simulink model "Task 2 – Battery Modeling"  (R2025b)
settings: Solver=ode23tb  StartTime=0.0  StopTime=35  RelTol=5e-3
model workspace (MAT data in the model file):
  Eng.Tbts = [18.9199441202 18.9199441202 24.2934146345 29.2101064979 38.0525747067 43.75 43.7497238015 43.7499913003 43.75 43.75 43.75 43.75 43.75 39.375 35 30.625]
  Eng.Nbts = [0 1500 2107.14285714 2714.28571429 3321.42857143 3928.57142857 4535.71428571 5142.85714286 5750 6357.14285714 6964.28571429 7571.42857143 8178.57142857 8785.71428571 9392.85714286 10000]
  Nmtr = 18.5
  SteerLim = 60
  TrackPoints = [-15 -12 -9 -6 -3 5.58745102111e-16 2.81978007367 5.36354042717 7.38228007367 8.67839071119 9.125 8.67839071119 ... (270 elements, 90x3)]
  Trans.InputShaftInertia = 0.01
  Trans.InputShaftDamping = 0.001
  Trans.FinalDrive = 3.25
  Trans.GearRatios = [-3.82 4.56 4.56 3.385 2.857 2.444 2 1]
  Trans.GearNums = [-1 0 1 2 3 4 5 6]
  Trans.Inertias = [0.032 0.007 0.032 0.025 0.0155 0.007 0.0025 0.0025]
  Trans.DampingCoeffs = [0.003 0.001 0.003 0.0025 0.002 0.001 0.001 0.001]
  Trans.Efficiencies = [0.9 0.9 0.9 0.9 0.9 0.95 0.95 0.95]
  Trans.ShiftTau = 0.02
  Ts = 0.02
  VEH.Mass = 230
  VEH.StaticNormalFrontLoad.FR = 575
  VEH.StaticNormalFrontLoad.FL = 575
  VEH.StaticNormalRearLoad.RR = 575
  VEH.StaticNormalRearLoad.RL = 322
  VEH.WheelBase = 1.7
  VEH.FrontAxlePositionfromCG = 0.75
  VEH.RearAxlePositionfromCG = 0.75
  VEH.HeightCG = 0.25
  VEH.FrontalArea = 2.11
  VEH.DragCoefficient = 0.33
  VEH.NumberOfWheelsPerAxle = 2
  VEH.PitchMomentInertia = 384.533333333
  VEH.RollMomentInertia = 86.4666666667
  VEH.YawMomentInertia = 413.2
  VEH.SteeringRatio = 18
  VEH.TrackWidth = 1.2
  VEH.SprungMass = 210
  VEH.InitialLongPosition = -15
  VEH.InitialLatPosition = 0
  VEH.InitialVertPosition = -0.2
  VEH.InitialRollAngle = 0
  VEH.InitialPitchAngle = 0
  VEH.InitialYawAngle = 0
  VEH.InitialLongVel = 0
  VEH.InitialLatVel = 0
  VEH.InitialVertVel = 0
  VEH.InitialRollRate = 0
  VEH.InitialPitchRate = 0
  VEH.InitialYawRate = 0
undefined symbols (not defined in the file or in its folder): BdyFrm, InertFrm
libraries: autolibsharedcoupling x11, simulink x9, sim3dlib x7, autolibutils x5, autolibshareddiff x5, sim3dautolib x3, vehdynlibtirecommon x3, sharedtransform x3, vehdynlibdriver x2, vehdynlibviscommon x2, vehdynlibtire x1, autolibmappedmotor x1
(part 1 of 4)
settings Model: SimulationMode=accelerator  Creator=The MathWorks, Inc.
settings SolverCC: ZeroCrossAlgorithm=Adaptive
settings OptimizationCC: ReuseModelBlockBuffer=off
settings DebuggingCC: IgnoredZcDiagnostic=none  SubsystemReferenceDiagnosticForUnitTest=warning
settings RTWCC: GPUComputeCapability=3.5

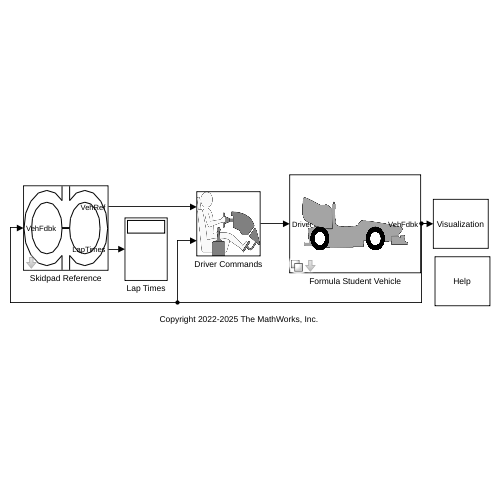
[thumbnail: Simulink's stored preview of the top-level diagram]
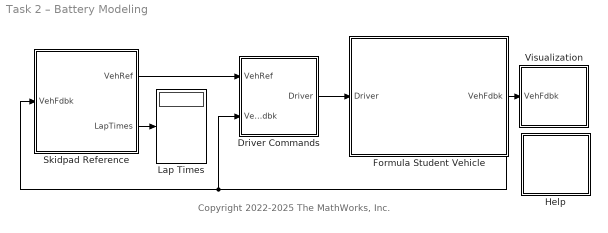
== system Task 2 – Battery Modeling ==
  note: Copyright 2022-2025 The MathWorks, Inc.
  Driver Commands : Subsystem  VariantControl=0
      mask Display: image('driverlatlongshift.png');
  Formula Student Vehicle : Subsystem  Variant=on  VariantControl=Choice  mask(Vehicle Setup){vehType=Simulink Physics}
      mask prompts: vehType "Vehicle Type:"
      mask help:
      | Choose a vehicle with powertrain and vehicle physics from Simulink blocks or one that uses a game engine physics.
      | The model will automatically configure the subsystems and settings to accomodate your choice.
      mask Help: eval('vdynblkshelp(''vdynblksformula'')');
      mask TypeOptions vehType: Game Engine Physics | Simulink Physics
      mask Callback vehType:
      | if strcmp(get_param(gcb,"vehType"),"Game Engine Physics")
      |     set_param([bdroot(gcs) '/Visualization/3D Visualization'],'engine3D','Enabled - Game Physics Vehicle')
      | else
      |     if strcmp(get_param([bdroot(gcs) '/Visualization/3D Visualization'],'engine3D'),'Enabled - Game Physics Vehicle')
      |         set_param([bdroot(gcs) '/Visualization/3D Visualization'],'engine3D','Enabled - Simulink 3D Vehicle')
      |     end
      | end
      mask Display: image('$imagefile'); % Use "Edit Image" on toolstrip to change.
  Help : Subsystem
      settings: OpenFcn=eval('vdynblkshelp(''vdynblksformula'')');
      mask Display: disp('Help')
  Lap Times : Display
  Skidpad Reference : Subsystem
      mask Display:
      | entryWidth = 3.453;
      | hOffset = 40;
      | vOffset = 15;
      | offset = [40,15];
      | entryConesLocR = [entryWidth/2 -12; entryWidth/2 -7.939];
      | entryConesLocL = [-entryWidth/2 -12;-entryWidth/2 -7.939];
      | plot(entryConesLocR(:,1)+hOffset,entryConesLocR(:,2)+vOffset);
      | plot(entryConesLocL(:,1)+hOffset,entryConesLocL(:,2)+vOffset);
      | 
      | rightInnerRingLoc = [entryWidth/2 0;...%1
      |                   4.58/2 -2.834;...%2
      |                   7.787/2 -5.231;...%3
      |                   12.588/2 -6.835;...%4
      |                   18.25/2 -7.398;...%5
      |                   23.912/2 -6.835;...%6
      |                   28.713/2 -5.231;...%7
      |                   31.92/2 -2.834;...%8
      |                   33.047/2 0;...%9
      |                   31.92/2 2.834;...%10
      |                   28.713/2 5.231;...%11
      |                   23.912/2 6.835;...%12
      |                   18.25/2 7.398;...%13
      |                   12.588/2 6.835;...%14
      |                   7.787/2 5.231;...%15
      |                   4.58/2 2.834;...%16
      |                   entryWidth/2 0;];
      | plot(rightInnerRingLoc(:,1)+hOffset,rightInnerRingLoc(:,2)+vOffset);
      | 
      | leftInnerRingLoc = rightInnerRingLoc.*[-1 1];
      | plot(leftInnerRingLoc(:,1)+hOffset,leftInnerRingLoc(:,2)+vOffset);
      | 
      | rightOutterRingLoc = [entryWidth/2 7.939;...
      |                       9.945/2 10.026;...
      |                       18.25/2 10.852;...
      |                       26.555/2 10.026;...
      |                       33.596/2 7.673;...
      |                       38.301/2 4.153;...
      |                       39.953/2 0;...
      |                       38.301/2 -4.153;...
      |                       33.596/2 -7.673;...
      |                       26.555/2 -10.026;...
      |                       18.25/2 -10.852;...
      |                       9.945/2 -10.026;...
      |                       entryWidth/2 -7.939];
      | plot(rightOutterRingLoc(:,1)+hOffset,rightOutterRingLoc(:,2)+vOffset);
      | leftOutterRingLoc = rightOutterRingLoc.*[-1 1];
      | plot(leftOutterRingLoc(:,1)+hOffset,leftOutterRingLoc(:,2)+vOffset);
      | exitConesLocL = entryConesLocL.*[1 -1];
      | exitConesLocR = entryConesLocR.*[1 -1];
      | plot(exitConesLocL(:,1)+hOffset,exitConesLocL(:,2)+vOffset);
      | plot(exitConesLocR(:,1)+hOffset,exitConesLocR(:,2)+vOffset);
      | plot([-1 1].*entryWidth/2+hOffset,[.1 .1]+vOffset)
      | plot([-1 1].*entryWidth/2+hOffset,[-.1 -.1]+vOffset)
  Visualization : Subsystem
      mask Display: disp('Visualization')
  wires:
  Driver Commands/1(Driver) -> Formula Student Vehicle/1(Driver)
  Skidpad Reference/1(VehRef) -> Driver Commands/1(VehRef)
  Formula Student Vehicle/1(VehFdbk) -> Driver Commands/2(VehFdbk), Skidpad Reference/1(VehFdbk), Visualization/1(VehFdbk)
  Skidpad Reference/2(LapTimes) -> Lap Times/1

== system Task 2 – Battery Modeling/Driver Commands ==
  VehRef : Inport
  VehFdbk : Inport  Port=2
  Bus Creator2 : BusCreator  Inputs=6
  Bus Selector3 : BusSelector  OutputSignals=VehFdbk.BdyFrm.Cg.Vel.xdot,VehFdbk.InertFrm.Cg.Disp.X,VehFdbk.InertFrm.Cg.Disp.Y,VehFdbk.InertFrm.Cg.Ang.psi,VehFdbk.BdyFrm.Cg.AngVel.r
  Bus Selector4 : BusSelector  OutputSignals=LngRef,PoseRef,EnblSteerCmd,SteerOvrCmd,SteerHld,SteerZero,EnblAccelOvr,AccelOvrCmd,AccelHld,AccelZero,EnblDecelCmd,DecelOvrCmd,DecelHld,DecelZero,CurvRef
  Constant1 : Constant  Value=0
  Ground1 : Ground
  Linear Predictive Driver : vehdynlibdriver/Predictive Driver  extAccelOvr=on  extDecelOvr=on  extAccelHld=on  extDecelHld=on  extAccelZero=on  extDecelZero=on  extSteerOvr=on  extSteerHld=on  extSteerZero=on  cntrlType=Predictive  cntrlTypeLat=Stanley  shftType=Scheduled  coordMode=SAE J670 (Z-down)  refType=Reference pose  velUnits=km/h  angUnits=rad  gearOut=on  steerOut=off  Kp=3  Ki=1  Kff=1  Kg=0  VehVelVec=[0 100]  KffVec=[.1 .1]  KpVec=[10 10]  KiVec=[5 5]  KgVec=[0 0]  vnom=5  Kaw=1  tauerr=.075  tau=.1  L=6  Kpt=8000  aR=200  bR=2.5  cR=.5  g=9.81  vecPose=on  dynamMode=on  PositionGainF=2.5  PositionGainR=.5  YawRateGain=.1  DelayGain=.01  enableDrift=off  BetaRef=10  KpBeta=1  KpDrift=1  KdDrift=1  KpPsi=1  KOmega=.1  tOmega=.1  a=VEH.FrontAxlePositionfromCG  b=VEH.RearAxlePositionfromCG  m=VEH.Mass  Cy_f=75000  Cy_r=70000  I=VEH.YawMomentInertia  Ksteer=1  theta=SteerLim*pi/180  Idl=1  Re=.3  lambda_mu=1  GearInit=0  tShift=.1  pdlVec=[0.1 0.4 0.5 0.9]  upShftTbl=[-1 12.9375 26.4375 39.9375 51.18749999999999 62.4375 72.84375 83.25;-1 16.3125 29.8125 43.3125 54.5624 65.8125 76.78125 87.75;-1 19.6875 33.1875 46.68749999999999 57.9375 69.1875 80.71875 92.25;-1 33 52.5 77.25 100.5 138.75 161.875 185]./2  dwnShftTbl=[-1 12.9375 26.4375 39.9375 51.18749999999999 62.4375 72.84375 83.25;-1 16.3125 29.8125 43.3125 54.5624 65.8125 76.78125 87.75;-1 19.6875 33.1875 46.68749999999999 57.9375 69.1875 80.71875 92.25;-1 33 52.5 77.25 100.5 138.75 161.875 185]./4  tClutch=.1  tRev=.5  tPark=120  UpGearVec="[0  1  2  3  4  5  6  7]"  DownGearVec="[1  2  3  4  5  6  7  8]"  aMode=2
  Mux1 : Mux  Inputs=3
  Mux2 : Mux  Inputs=2
  Selector1 : Selector  InputPortWidth=3  IndexOptions=Index vector (dialog)  Indices=[1 2]  OutputSizes=1
  Subsystem : Subsystem
  Terminator1 : Terminator
  Unit Conversion : UnitConversion
  Driver : Outport  VectorParamsAs1DForOutWhenUnconnected=off
  wires:
  Linear Predictive Driver/4 -> Bus Creator2/3, Subsystem/1(DecelCmd)  "DecelCmd"
  Linear Predictive Driver/2 -> Bus Creator2/1  "SteerCmd"
  Bus Creator2/1 -> Driver/1
  Linear Predictive Driver/3 -> Bus Creator2/2  "AccelCmd"
  Linear Predictive Driver/5 -> Subsystem/2(GearCmd), Bus Creator2/4  "GearCmd"
  Bus Selector4/9 -> Linear Predictive Driver/9  "<AccelHld>"
  Ground1/1 -> Linear Predictive Driver/15
  Bus Selector3/1 -> Unit Conversion/1  "<xdot>"
  Bus Selector4/13 -> Linear Predictive Driver/13  "<DecelHld>"
  Bus Selector4/14 -> Linear Predictive Driver/14  "<DecelZero>"
  Bus Selector4/7 -> Linear Predictive Driver/7  "<EnblAccelOvr>"
  Bus Selector4/11 -> Linear Predictive Driver/11  "<EnblDecelCmd>"
  Bus Selector4/1 -> Linear Predictive Driver/1  "<LngRef>"
  Bus Selector4/12 -> Linear Predictive Driver/12  "<DecelOvrCmd>"
  Bus Selector4/8 -> Linear Predictive Driver/8  "<AccelOvrCmd>"
  Bus Selector4/4 -> Linear Predictive Driver/4  "<SteerOvrCmd>"
  Bus Selector4/10 -> Linear Predictive Driver/10  "<AccelZero>"
  Bus Selector4/5 -> Linear Predictive Driver/5  "<SteerHld>"
  Bus Selector4/6 -> Linear Predictive Driver/6  "<SteerZero>"
  Bus Selector4/3 -> Linear Predictive Driver/3  "<EnblSteerCmd>"
  Linear Predictive Driver/1 -> Terminator1/1
  VehFdbk/1 -> Bus Selector3/1
  VehRef/1 -> Bus Selector4/1
  Bus Selector3/4 -> Mux1/3  "<psi>"
  Bus Selector3/2 -> Mux1/1  "<X>"
  Bus Selector3/3 -> Mux1/2  "<Y>"
  Subsystem/1(Light controls) -> Bus Creator2/5  "Light controls"
  Bus Selector4/2 -> [PoseRef], Linear Predictive Driver/2  "<PoseRef>"
  Mux1/1 -> Linear Predictive Driver/18  "Ref"
  Selector1/1 -> Mux2/1
  [PoseRef] -> Selector1/1
  Constant1/1 -> Mux2/2
  Mux2/1 -> Bus Creator2/6  "Ref"
  Unit Conversion/1 -> Linear Predictive Driver/17
  Bus Selector4/15 -> Linear Predictive Driver/16  "<CurvRef>"
  Bus Selector3/5 -> Linear Predictive Driver/19  "<r>"

== system Task 2 – Battery Modeling/Formula Student Vehicle ==
  Driver : Inport
  Game Engine Physics : Subsystem  VariantControl=vehType==1
  Simulink Physics - 7DOF : Subsystem  VariantControl=vehType==2
  VehFdbk : Outport

== system Task 2 – Battery Modeling/Help ==

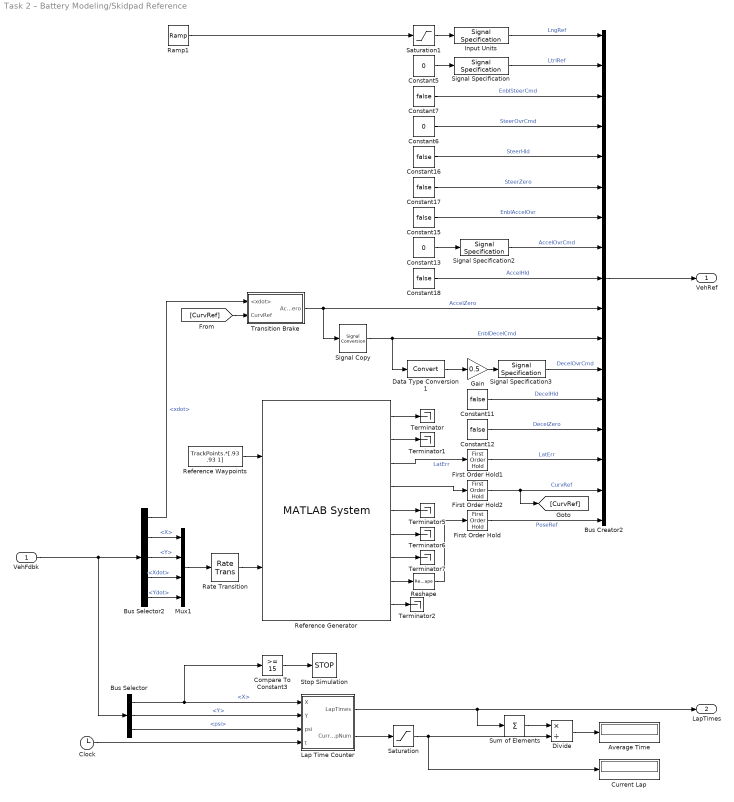
== system Task 2 – Battery Modeling/Skidpad Reference ==
  VehFdbk : Inport
  Average Time : Display
  Bus Creator2 : BusCreator  Inputs=17
  Bus Selector : BusSelector  OutputSignals=VehFdbk.InertFrm.Cg.Disp.X,VehFdbk.InertFrm.Cg.Disp.Y,VehFdbk.InertFrm.Cg.Ang.psi
  Bus Selector2 : BusSelector  OutputSignals=VehFdbk.BdyFrm.Cg.Vel.xdot,VehFdbk.InertFrm.Cg.Disp.X,VehFdbk.InertFrm.Cg.Disp.Y,VehFdbk.InertFrm.Cg.Vel.Xdot,VehFdbk.InertFrm.Cg.Vel.Ydot
  Clock : Clock
  Compare To Constant3 : simulink/Logic and Bit Operations/Compare To Constant  relop=>=  const=15  OutDataTypeStr=boolean  ZeroCross=off
  Constant{11..12,15..18} (6 alike) : Constant  Value=false
  Constant13 : Constant  Value=0
  Constant5 : Constant  Value=0
  Constant6 : Constant  Value=0
  Constant7 : Constant  Value=false  OutDataTypeStr=boolean
  Current Lap : Display
  Data Type Conversion1 : DataTypeConversion  SaturateOnIntegerOverflow=off  RndMeth=Floor
  Divide : Product  Inputs=*/
  First Order Hold : FirstOrderHold  InitialOutput=[VEH.InitialLongPosition VEH.InitialLatPosition VEH.InitialYawAngle]  ErrorTolerance=.1
  First Order Hold1 : FirstOrderHold  ErrorTolerance=.1
  First Order Hold2 : FirstOrderHold  ErrorTolerance=.1
  Gain : Gain  Gain=0.5
  Input Units : SignalSpecification  Unit=km/h
  Lap Time Counter : MATLAB Function  TreatAsAtomicUnit=on
  Mux1 : Mux
  Ramp1 : simulink/Sources/Ramp  slope=5  start=2  InitialOutput=0
  Rate Transition : RateTransition  InitialCondition=[VEH.InitialLongPosition VEH.InitialLatPosition 0 0]  OutPortSampleTime=Ts
  Reference Generator : vehdynlibdriver/Predictive Driver/Pose Routing/XY Waypoints Vector/MATLAB System  ShowRefPath=off  arcLengthHorizon=10  RollingSegment=off  SegLen=1000  LoopTrajectory=off  numOfHrzPoints=20  SimulateUsing=Interpreted execution
  Reference Waypoints : Constant  Value=TrackPoints.*[.93 .93 1]
  Reshape : Reshape
  Saturation : Saturate  UpperLimit=6  LowerLimit=1  ZeroCross=off
  Saturation1 : Saturate  UpperLimit=39.0  LowerLimit=0  ZeroCross=off
  Signal Copy : SignalConversion  OverrideOpt=off
  Signal Specification : SignalSpecification  Unit=m
  Signal Specification2 : SignalSpecification  Unit=one
  Signal Specification3 : SignalSpecification  Unit=one
  Stop Simulation : Stop
  Sum of Elements : Sum  Inputs=+
  Terminator{,1..2,5..7} (6 alike) : Terminator
  Transition Brake : Subsystem
  VehRef : Outport
  LapTimes : Outport  Port=2
  wires:
  Saturation1/1 -> Input Units/1
  Constant13/1 -> Signal Specification2/1
  Signal Specification/1 -> Bus Creator2/2  "LtrlRef"
  Constant7/1 -> Bus Creator2/3  "EnblSteerCmd"
  Constant11/1 -> Bus Creator2/13  "DecelHld"
  Reference Generator/7 -> Terminator7/1
  Reference Generator/8 -> Reshape/1
  Reference Generator/5 -> Terminator5/1
  Reference Generator/2 -> Terminator1/1
  Reference Generator/4 -> First Order Hold2/1
  Reference Generator/6 -> Terminator6/1
  Constant16/1 -> Bus Creator2/5  "SteerHld"
  VehFdbk/1 -> Bus Selector/1, Bus Selector2/1
  Signal Copy/1 -> Data Type Conversion1/1, Bus Creator2/11  "EnblDecelCmd"
  Constant5/1 -> Signal Specification/1
  Constant17/1 -> Bus Creator2/6  "SteerZero"
  Reference Generator/9 -> Terminator2/1
  First Order Hold1/1 -> Bus Creator2/15  "LatErr"
  Input Units/1 -> Bus Creator2/1  "LngRef"
  Bus Creator2/1 -> VehRef/1
  Ramp1/1 -> Saturation1/1
  Constant18/1 -> Bus Creator2/9  "AccelHld"
  Signal Specification2/1 -> Bus Creator2/8  "AccelOvrCmd"
  Signal Specification3/1 -> Bus Creator2/12  "DecelOvrCmd"
  Reference Generator/1 -> Terminator/1
  Constant12/1 -> Bus Creator2/14  "DecelZero"
  Constant15/1 -> Bus Creator2/7  "EnblAccelOvr"
  Constant6/1 -> Bus Creator2/4  "SteerOvrCmd"
  Bus Selector2/4 -> Mux1/3  "<Xdot>"
  Bus Selector2/2 -> Mux1/1  "<X>"
  Bus Selector2/5 -> Mux1/4  "<Ydot>"
  Mux1/1 -> Rate Transition/1
  Bus Selector2/3 -> Mux1/2  "<Y>"
  Reshape/1 -> First Order Hold/1
  Bus Selector/1 -> Compare To Constant3/1, Lap Time Counter/1(X)  "<X>"
  Bus Selector/2 -> Lap Time Counter/2(Y)  "<Y>"
  Bus Selector/3 -> Lap Time Counter/3(psi)  "<psi>"
  Clock/1 -> Lap Time Counter/4(t)
  Lap Time Counter/1(LapTimes) -> Sum of Elements/1, LapTimes/1
  Reference Waypoints/1 -> Reference Generator/1
  Data Type Conversion1/1 -> Gain/1
  Gain/1 -> Signal Specification3/1
  Rate Transition/1 -> Reference Generator/2
  First Order Hold/1 -> Bus Creator2/17  "PoseRef"
  Reference Generator/3 -> First Order Hold1/1  "LatErr"
  First Order Hold2/1 -> [CurvRef], Bus Creator2/16  "CurvRef"
  Transition Brake/1(AccelZero) -> Signal Copy/1, Bus Creator2/10  "AccelZero"
  Bus Selector2/1 -> Transition Brake/1(<xdot>)  "<xdot>"
  Compare To Constant3/1 -> Stop Simulation/1
  Lap Time Counter/2(CurrLapNum) -> Saturation/1
  Sum of Elements/1 -> Divide/1
  Divide/1 -> Average Time/1
  Saturation/1 -> Current Lap/1, Divide/2
  [CurvRef] -> Transition Brake/2(CurvRef)

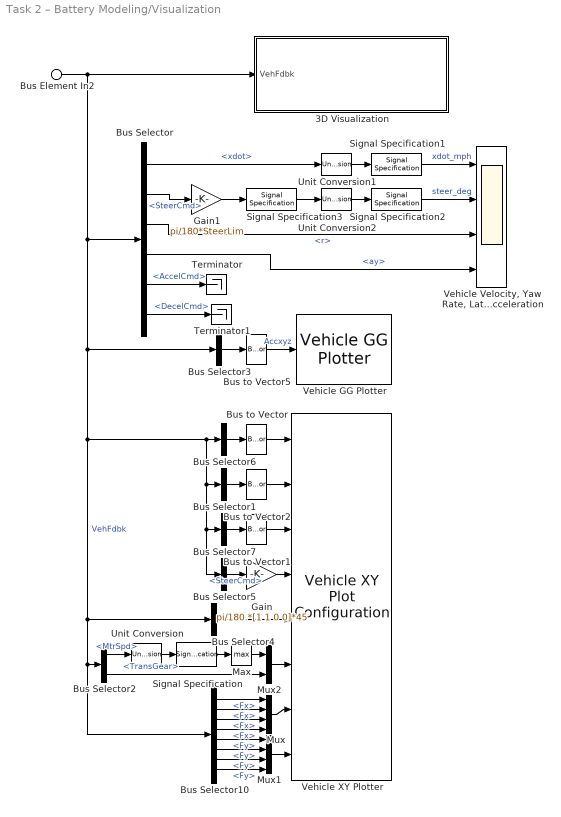
== system Task 2 – Battery Modeling/Visualization ==
  Bus Element In2 : Inport  PortName=VehFdbk
  3D Visualization : Subsystem  Variant=on  VariantControl=Choice  mask(3D Visualization Setup){engine3D=Disabled, conesOn=on, annotOn=on, pathOn=on, InitialPos=[ VEH.InitialLongPosition, VEH.InitialLatPosition, VEH.InitialVertPosition ], InitialRot=[VEH.InitialRollAngle VEH.InitialPitchAngle VEH.InitialYawAngle], Ts=Ts}
      mask prompts: engine3D "Visualization Mode:"; conesOn "Include cones"; annotOn "Include annotations"; pathOn "Include path markers"; InitialPos "shared_sim3dblks:sim3dblkVehicleWithGroundFollowingVDBS:blkPrm_InitialPos"; InitialRot "shared_sim3dblks:sim3dblkVehicleWithGroundFollowingVDBS:blkPrm_InitialRotSAE"; Ts "shared_sim3dblks:sim3dblkConfig:Ts"
      mask help: This is an example specific block designed to only work with vydnblksskidpad.slx. It is used in conjuction with the vehicle subystem to provide options for the 3D game engine visualization (requires Simulink 3D Animation).
      mask init:
      | visType = get_param(gcb,"engine3D");
      | switch visType
      |     case "Disabled"
      |         autoblksenableparameters(gcb, [],{'conesOn';'annotOn';'pathOn'},[],[],true);
      |         set_param([bdroot '/Formula Student Vehicle'],'vehType','Simulink Physics')
      |     case "Enabled - Ground Following Vehicle"
      |         set_param([bdroot '/Formula Student Vehicle'],'vehType','Simulink Physics')
      |         autoblksenableparameters(gcb, {'conesOn';'annotOn';'pathOn'},[],[],[],true);
      |     case "Enabled - Game Physics Vehicle"
      |         set_param([bdroot '/Formula Student Vehicle'],'vehType','Game Engine Physics')
      |         autoblksenableparameters(gcb, {'conesOn';'annotOn';'pathOn'},[],[],[],true);
      | end
      settings: AttributesFormatString=%<engine3D>
      mask TypeOptions engine3D: Disabled | Enabled - Simulink 3D Vehicle | Enabled - Game Physics Vehicle
      mask Callback engine3D:
      | if strcmp(get_param(gcb,"engine3D"),"Disabled")
      |     autoblksenableparameters(gcb, [],{'conesOn';'annotOn';'pathOn'},[],[],true);
      | else
      |     autoblksenableparameters(gcb, {'conesOn';'annotOn';'pathOn'},[],[],[],true);
      | end
      mask DialogControl InitialPos Prompt: Initial position [X, Y, Z], InitialPos [m]:
      mask DialogControl InitialRot Prompt: Initial rotation [Roll, Pitch, Yaw], InitialRot [rad]:
      mask DialogControl Ts Prompt: Sample time:
  Bus Selector : BusSelector  OutputSignals=VehFdbk.BdyFrm.Cg.Vel.xdot,Driver.SteerCmd,VehFdbk.BdyFrm.Cg.AngVel.r,VehFdbk.BdyFrm.Cg.Acc.ay,Driver.AccelCmd,Driver.DecelCmd
  Bus Selector1 : BusSelector  OutputSignals=VehFdbk.InertFrm.Cg.Ang.phi,VehFdbk.InertFrm.Cg.Ang.theta,VehFdbk.InertFrm.Cg.Ang.psi  OutputAsBus=on
  Bus Selector10 : BusSelector  OutputSignals=VehFdbk.BdyFrm.Forces.Tires.FrntTires.Lft.Fx,VehFdbk.BdyFrm.Forces.Tires.FrntTires.Rght.Fx,VehFdbk.BdyFrm.Forces.Tires.RearTires.Lft.Fx,VehFdbk.BdyFrm.Forces.Tires.RearTires.Rght.Fx,VehFdbk.BdyFrm.Forces.Tires.FrntTires.Lft.Fy,VehFdbk.BdyFrm.Forces.Tires.FrntTires.Rght.Fy,VehFdbk.BdyFrm.Forces.Tires.RearTires.Lft.Fy,VehFdbk.BdyFrm.Forces.Tires.RearTires.Rght.Fy
  Bus Selector2 : BusSelector  OutputSignals=VehFdbk.Mtr.MtrSpd,VehFdbk.Trans.TransGear
  Bus Selector3 : BusSelector  OutputSignals=VehFdbk.BdyFrm.Cg.Acc.ax,VehFdbk.BdyFrm.Cg.Acc.ay,VehFdbk.BdyFrm.Cg.Acc.az  OutputAsBus=on
  Bus Selector4 : BusSelector  OutputSignals=Driver.Ref  OutputAsBus=on
  Bus Selector5 : BusSelector  OutputSignals=Driver.SteerCmd
  Bus Selector6 : BusSelector  OutputSignals=VehFdbk.InertFrm.Cg.Disp.X,VehFdbk.InertFrm.Cg.Disp.Y,VehFdbk.InertFrm.Cg.Disp.Z  OutputAsBus=on
  Bus Selector7 : BusSelector  OutputSignals=VehFdbk.InertFrm.Cg.Vel.Xdot,VehFdbk.InertFrm.Cg.Vel.Ydot,VehFdbk.InertFrm.Cg.Vel.Zdot  OutputAsBus=on
  Bus to Vector{,1..2,5} (4 alike) : BusToVector
  Gain : Gain  Gain=pi/180.*[1 1 0 0]*45
  Gain1 : Gain  Gain=pi/180*SteerLim
  Max : MinMax  Function=max  ZeroCross=off
  Mux : Mux
  Mux1 : Mux
  Mux2 : Mux  Inputs=2
  Signal Specification : SignalSpecification  Unit=rad/s
  Signal Specification1 : SignalSpecification  Unit=mph
  Signal Specification2 : SignalSpecification  Unit=deg
  Signal Specification3 : SignalSpecification  Unit=rad
  Terminator : Terminator
  Terminator1 : Terminator
  Unit Conversion : UnitConversion
  Unit Conversion1 : UnitConversion
  Unit Conversion2 : UnitConversion
  Vehicle GG Plotter : vehdynlibviscommon/Vehicle GG Plotter  axesType=+z down, inertial  gScale=2  pltDT=.1
  "Vehicle Velocity, Yaw Rate, Lateral Acceleration" : Scope  NumInputPorts=4
      settings: ActiveDisplayYMinimum=-3.35522  ActiveDisplayYMaximum=27.7947
  Vehicle XY Plotter : vehdynlibviscommon/Vehicle XY Plot Configuration  extRef=on  extStats=on  extTireF=on  a=VEH.FrontAxlePositionfromCG  b=VEH.RearAxlePositionfromCG  w=VEH.TrackWidth  figBorder=10  bufferSize=2048  velNorm=10  tireFNorm=1000  pltDT=.2
  wires:
  Bus Selector7/1 -> Bus to Vector1/1
  Bus to Vector/1 -> Vehicle XY Plotter/1
  Bus Selector6/1 -> Bus to Vector/1
  Bus to Vector1/1 -> Vehicle XY Plotter/3
  Bus Selector1/1 -> Bus to Vector2/1
  Bus Element In2/1 -> 3D Visualization/1(VehFdbk), Bus Selector3/1, Bus Selector10/1, Bus Selector2/1, Bus Selector4/1, Bus Selector5/1, Bus Selector7/1, Bus Selector1/1, Bus Selector6/1, Bus Selector/1  "VehFdbk"
  Bus to Vector2/1 -> Vehicle XY Plotter/2
  Bus Selector5/1 -> Gain/1  "<SteerCmd>"
  Unit Conversion1/1 -> Signal Specification1/1
  Bus Selector/4 -> "Vehicle Velocity, Yaw Rate, Lateral Acceleration"/4  "<ay>"
  Bus Selector/1 -> Unit Conversion1/1  "<xdot>"
  Signal Specification1/1 -> "Vehicle Velocity, Yaw Rate, Lateral Acceleration"/1  "xdot_mph"
  Bus Selector/3 -> "Vehicle Velocity, Yaw Rate, Lateral Acceleration"/3  "<r>"
  Bus Selector4/1 -> Vehicle XY Plotter/5
  Gain/1 -> Vehicle XY Plotter/4
  Mux2/1 -> Vehicle XY Plotter/6
  Bus Selector2/2 -> Mux2/2  "<TransGear>"
  Bus Selector/2 -> Gain1/1  "<SteerCmd>"
  Unit Conversion2/1 -> Signal Specification2/1
  Signal Specification2/1 -> "Vehicle Velocity, Yaw Rate, Lateral Acceleration"/2  "steer_deg"
  Bus to Vector5/1 -> Vehicle GG Plotter/1  "Accxyz"
  Bus Selector3/1 -> Bus to Vector5/1
  Mux/1 -> Vehicle XY Plotter/7
  Mux1/1 -> Vehicle XY Plotter/8
  Bus Selector10/1 -> Mux/1  "<Fx>"
  Bus Selector10/2 -> Mux/2  "<Fx>"
  Bus Selector10/3 -> Mux/3  "<Fx>"
  Bus Selector10/4 -> Mux/4  "<Fx>"
  Bus Selector10/5 -> Mux1/1  "<Fy>"
  Bus Selector10/6 -> Mux1/2  "<Fy>"
  Bus Selector10/7 -> Mux1/3  "<Fy>"
  Bus Selector10/8 -> Mux1/4  "<Fy>"
  Gain1/1 -> Signal Specification3/1
  Signal Specification3/1 -> Unit Conversion2/1
  Unit Conversion/1 -> Signal Specification/1
  Bus Selector2/1 -> Unit Conversion/1  "<MtrSpd>"
  Signal Specification/1 -> Max/1
  Bus Selector/5 -> Terminator/1  "<AccelCmd>"
  Bus Selector/6 -> Terminator1/1  "<DecelCmd>"
  Max/1 -> Mux2/1

== system Task 2 – Battery Modeling/Driver Commands/Subsystem ==
  note: Light Logic
  DecelCmd : Inport
  GearCmd : Inport  Port=2
  Brake : simulink/Logic and Bit Operations/Compare To Constant  relop=>  const=.01  OutDataTypeStr=boolean  ZeroCross=off
  Highbeam : Constant  Value=false
  Left Signal : Constant  Value=false
  Lowbeam : Constant  Value=false
  Mux1 : Mux  Inputs=6
  Reverse : simulink/Logic and Bit Operations/Compare To Constant  relop=<  const=0  OutDataTypeStr=boolean  ZeroCross=off
  Right Signal : Constant  Value=false
  Light controls : Outport
  wires:
  Brake/1 -> Mux1/3
  DecelCmd/1 -> Brake/1
  Highbeam/1 -> Mux1/1
  Right Signal/1 -> Mux1/6
  Left Signal/1 -> Mux1/5
  Lowbeam/1 -> Mux1/2
  Reverse/1 -> Mux1/4
  Mux1/1 -> Light controls/1
  GearCmd/1 -> Reverse/1

== system Task 2 – Battery Modeling/Formula Student Vehicle/Game Engine Physics ==
  note: Vehicle Dynamics - Game Engine Physics
      | This block provides a signal and parameter interface such that a complete vehicle can be simulated and visualized with the game engine, including rigid body collision and ground contact.
  Driver : Inport
  Bus Assignment : BusAssignment  AssignedSignals=BdyFrm.Cg.Vel.xdot,InertFrm.Cg.Disp.X,InertFrm.Cg.Disp.Y,InertFrm.Cg.Ang.psi
  Bus Creator : BusCreator  Inputs=2
  Bus Selector : BusSelector  OutputSignals=SteerCmd,AccelCmd,DecelCmd,GearCmd,Light controls
  Bus Selector1 : BusSelector  OutputSignals=BdyFrm.Cg.Vel.xdot,InertFrm.Cg.Disp.X,InertFrm.Cg.Disp.Y,InertFrm.Cg.Ang.psi
  First Order Hold : FirstOrderHold  ErrorTolerance=.1
  First Order Hold1 : FirstOrderHold  InitialOutput=VEH.InitialLongPosition  ErrorTolerance=.1
  First Order Hold2 : FirstOrderHold  InitialOutput=VEH.InitialLatPosition  ErrorTolerance=.1
  First Order Hold6 : FirstOrderHold  InitialOutput=VEH.InitialYawAngle  ErrorTolerance=.01
  Rate Transition : RateTransition
  Simulation 3D Physics Vehicle : sim3dautolib/Simulation 3D Physics Vehicle  Priority=-1  PassVehMesh=Formula student vehicle  VehColor=Red  ActorName=SimulinkVehicle2  MeshPath=/MathWorksSimulation/Vehicles/Muscle/Meshes/SK_MuscleCar.SK_Sedan  TrackWidth=2  WheelBase=3  FrntWhlRadius=0.30  RearWhlRadius=0.30  FrntWhlWidth=0.20  RearWhlWidth=0.20  InitialPos=[ VEH.InitialLongPosition, VEH.InitialLatPosition, VEH.InitialVertPosition]  InitialRot=[VEH.InitialRollAngle VEH.InitialPitchAngle VEH.InitialYawAngle]  Mass=VEH.SprungMass  CgOffset=[ -.1, -.11, 0 ]  IvehScale=[1 1 1]  ChassisHeight=.5  Cd=0.2  Cl=0.1  TrqCrv=Eng.Tbts  SpdCrv=Eng.Nbts  MaxRPM=max(Eng.Nbts)  Jmot=.02  bEngMax=.025  bEngMin=.05  DrivetrainType=Rear Wheel Drive  FrontRearSplit=0.5  TransType=Manual  G=Trans.GearNums  N=Trans.GearRatios  UpShiftRPM=4000  DownShiftRPM=2000  MinRPM=750  tShift=.02  NDiff=Trans.FinalDrive  eta=0.94  SteerType=Ackermann  SteerAngleRatio=1.0  EnableFrontSteer=on  FrntWhlMaxSteer=6*pi/180*SteerLim  EnableRearSteer=off  RearWhlMaxSteer=0  SteerSpdFctTbl=[ 1,.9, .8]  SteerVehSpdBpts=[ 0, 60, 120 ]./3.6  FrntWhlMaxTrq=5  RearWhlMaxTrq=5  HndBrkEnable=off  FrntWhlHndBrkEnable=off  RearWhlHndBrkEnable=off  FrntWhlMaxHndBrkTrq=3000  RearWhlMaxHndBrkTrq=1500  FrntSuspFOffset=[0 0 0]  RearSuspFOffset=[0 0 0]  FrntSuspMaxComp=.1  RearSuspMaxComp=.1  FrntSpringPreload=200  RearSpringPreload=200  FrntSpringRate=7e3  RearSpringRate=7e3  FrntSuspMaxExt=.1  RearSuspMaxExt=.1  FrntSuspDamping=.25  RearSuspDamping=.25  FrntRollbarScaling=.5  RearRollbarScaling=.5  ABSEnable=off  TCSEnable=off  Cy_f=250e3  Cy_r=250e3  FrntSlipThreshold=.3  RearSlipThreshold=.3  FrntSkidThreshold=1.0  RearSkidThreshold=1.0  FrntSideSlipModifier=1  RearSideSlipModifier=1  ExtMu=off  lambda_mu=10  VehLightsControl=on  HeadlightColor=[ 1, 1, 1 ]  HighBeamIntensity=100000  LowBeamIntensity=60000  HighBeamConeAngle=1.22  LowBeamConeAngle=1.22  LeftHeadlightOrientation=[ 0, 0 ]  RightHeadlightOrientation=[ 0, 0 ]  BrakelightIntensity=500  ReverselightIntensity=500  SignallightIntensity=500  SignallightPeriod=1  SignalPulseWidth=50  StandardOutportEnabled=on  TransformOutportEnabled=off  SampleTime=Ts  ActorType=SimulinkVehicle  ID=2  aMode=2  ActorTag=SimulinkVehicle2  CoordinateScheme=SAE
      settings: LibrarySourceBlock=vdynlib/Vehicle Scenarios/Sim3D/Sim3D Vehicle/Components/Simulation 3D Physics Vehicle
  Terminator{,1..3} (4 alike) : Terminator
  VehFdbk : Outport
  wires:
  Driver/1 -> Bus Selector/1, Bus Creator/2  "Driver"
  Bus Creator/1 -> VehFdbk/1
  Bus Selector/2 -> Simulation 3D Physics Vehicle/2  "<AccelCmd>"
  Bus Selector/1 -> Simulation 3D Physics Vehicle/1  "<SteerCmd>"
  Bus Selector/4 -> Simulation 3D Physics Vehicle/4  "<GearCmd>"
  Bus Selector/3 -> Simulation 3D Physics Vehicle/3  "<DecelCmd>"
  Bus Assignment/1 -> Bus Creator/1  "VehFdbk"
  Simulation 3D Physics Vehicle/2 -> Terminator/1
  Simulation 3D Physics Vehicle/3 -> Terminator1/1
  Simulation 3D Physics Vehicle/4 -> Terminator2/1
  Simulation 3D Physics Vehicle/5 -> Terminator3/1
  Simulation 3D Physics Vehicle/1 -> Bus Selector1/1, Rate Transition/1
  Bus Selector1/1 -> First Order Hold/1  "<xdot>"
  Bus Selector1/2 -> First Order Hold1/1  "<X>"
  Bus Selector1/3 -> First Order Hold2/1  "<Y>"
  Rate Transition/1 -> Bus Assignment/1
  First Order Hold/1 -> Bus Assignment/2
  Bus Selector1/4 -> First Order Hold6/1  "<psi>"
  First Order Hold1/1 -> Bus Assignment/3
  First Order Hold2/1 -> Bus Assignment/4
  First Order Hold6/1 -> Bus Assignment/5
  Bus Selector/5 -> Simulation 3D Physics Vehicle/5  "<Light controls>"

== system Task 2 – Battery Modeling/Formula Student Vehicle/Simulink Physics - 7DOF ==
  note: Vehicle Dynamics
  Driver : Inport
  Bus Selector : BusSelector  OutputSignals=AccelCmd,DecelCmd,GearCmd
  Bus Selector1 : BusSelector  OutputSignals=Gnd.mu
  Bus Selector2 : BusSelector  OutputSignals=SteerCmd
  Bus Routing : Subsystem
  Environment : Subsystem
      mask Display: disp('Environment')
  Powertrain & Driveline : Subsystem
      mask Display: image('vdbslibpt.png');
  Steering : Subsystem
      mask Display: image('vdbslibsteer.png');
  Vehicle Body 3DOF Dual Track : Subsystem
      mask Display: image('3dofdtrack.png');
  VehFdbk : Outport
  wires:
  Vehicle Body 3DOF Dual Track/1(VehFdbk) -> Powertrain & Driveline/6(VehFdbk), Bus Routing/1(VehInfo)
  Powertrain & Driveline/2(Rear Force) -> Vehicle Body 3DOF Dual Track/3(FwR)
  Powertrain & Driveline/1(Front Force) -> Vehicle Body 3DOF Dual Track/2(FwF)
  Bus Selector/2 -> Powertrain & Driveline/3(Decel)  "<DecelCmd>"
  Steering/1(FrntWhl) -> Vehicle Body 3DOF Dual Track/1(WhlAngF)
  Powertrain & Driveline/3(Driveline) -> [Driveline]
  Bus Selector/3 -> Powertrain & Driveline/4(GearCmd)  "<GearCmd>"
  Bus Selector2/1 -> Powertrain & Driveline/1(HndWhl), Steering/1(HndWhl)  "<SteerCmd>"
  Bus Selector/1 -> Powertrain & Driveline/2(Acc)  "<AccelCmd>"
  Driver/1 -> Bus Selector2/1, [Driver], Bus Selector/1
  Environment/1(Env) -> Bus Selector1/1
  Bus Selector1/1 -> Powertrain & Driveline/5(Friction)  "<mu>"
  [Driver] -> Bus Routing/2(Driver)  "Driver"
  [Driveline] -> Bus Routing/3(Driveline)
  Bus Routing/1(VehFdbk) -> VehFdbk/1

== system Task 2 – Battery Modeling/Skidpad Reference/Transition Brake ==
  <xdot> : Inport
  CurvRef : Inport  Port=2
  Compare To Constant : simulink/Logic and Bit Operations/Compare To Constant  relop=>=  const=120  OutDataTypeStr=boolean  ZeroCross=off
  Compare To Constant1 : simulink/Logic and Bit Operations/Compare To Constant  relop=>=  const=0  OutDataTypeStr=boolean  ZeroCross=off
  Compare To Constant2 : simulink/Logic and Bit Operations/Compare To Constant  relop=<  const=260  OutDataTypeStr=boolean  ZeroCross=off
  Compare To Constant3 : simulink/Logic and Bit Operations/Compare To Constant  relop=>  const=5  OutDataTypeStr=boolean  ZeroCross=off
  Integrator : Integrator
  Logical Operator : Logic  Inputs=4  AllPortsSameDT=off  OutDataTypeStr=boolean
  AccelZero : Outport
  wires:
  Logical Operator/1 -> AccelZero/1
  Integrator/1 -> Compare To Constant2/1, Compare To Constant/1
  Compare To Constant2/1 -> Logical Operator/2
  Compare To Constant3/1 -> Logical Operator/1
  Compare To Constant/1 -> Logical Operator/3
  Compare To Constant1/1 -> Logical Operator/4
  <xdot>/1 -> Compare To Constant3/1, Integrator/1
  CurvRef/1 -> Compare To Constant1/1

== system Task 2 – Battery Modeling/Visualization/3D Visualization ==
  VehFdbk : Inport
  Disabled : Subsystem  VariantControl=engine3D==1
  Enabled : Subsystem  VariantControl=engine3D~=1

== system Task 2 – Battery Modeling/Formula Student Vehicle/Simulink Physics - 7DOF/Bus Routing ==
  VehInfo : Inport
  Driver : Inport  Port=2
  Driveline : Inport  Port=3
  Bus Creator : BusCreator  Inputs=2
  Bus Creator17 : BusCreator  Inputs=5
  Bus Creator3 : BusCreator  Inputs=2
  Bus Creator4 : BusCreator  Inputs=2
  Bus Selector3 : BusSelector  OutputSignals=MtrTrq,MtrSpd,TransGearCmd,TransGear,Wheels
  Bus Selector4 : BusSelector  OutputSignals=InertFrm,BdyFrm
  Signal Specification : SignalSpecification  Unit=rpm
  Signal Specification1 : SignalSpecification  Unit=one
  Signal Specification3 : SignalSpecification  Unit=one
  VehFdbk : Outport
  wires:
  Bus Selector3/2 -> Signal Specification/1  "<MtrSpd>"
  Bus Creator17/1 -> Bus Creator/2  "VehFdbk"
  Bus Selector3/1 -> Bus Creator3/1  "<MtrTrq>"
  Signal Specification3/1 -> Bus Creator4/1  "TransGearCmd"
  Bus Selector4/2 -> Bus Creator17/2  "<BdyFrm>"
  Bus Selector3/3 -> Signal Specification3/1  "<TransGearCmd>"
  Bus Selector3/4 -> Signal Specification1/1  "<TransGear>"
  Bus Selector4/1 -> Bus Creator17/1  "<InertFrm>"
  Bus Creator3/1 -> Bus Creator17/3  "Mtr"
  Bus Creator4/1 -> Bus Creator17/4  "Trans"
  Signal Specification1/1 -> Bus Creator4/2  "TransGear"
  Signal Specification/1 -> Bus Creator3/2  "MtrSpd"
  VehInfo/1 -> Bus Selector4/1
  Bus Creator/1 -> VehFdbk/1
  Driver/1 -> Bus Creator/1
  Driveline/1 -> Bus Selector3/1
  Bus Selector3/5 -> Bus Creator17/5  "<Wheels>"

== system Task 2 – Battery Modeling/Formula Student Vehicle/Simulink Physics - 7DOF/Environment ==
  Bus Creator2 : BusCreator  Inputs=2
  Constant1 : Constant  Value=0
  Constant2 : Constant  Value=0
  Constant3 : Constant  Value=ones(1,4)
  Constant6 : Constant  Value=0
  Ground Feedback : Subsystem  Variant=on  VariantControlMode=label  LabelModeActiveChoice=0
  Vector Concatenate1 : Concatenate  NumInputs=3
  Env : Outport  VectorParamsAs1DForOutWhenUnconnected=off
  wires:
  Ground Feedback/1(Ground) -> Bus Creator2/2  "Gnd"
  Vector Concatenate1/1 -> Bus Creator2/1  "Wind"
  Constant2/1 -> Vector Concatenate1/2  "Y"
  Bus Creator2/1 -> Env/1
  Constant6/1 -> Vector Concatenate1/3  "Z"
  Constant1/1 -> Vector Concatenate1/1  "X"
  Constant3/1 -> Ground Feedback/1(Friction)

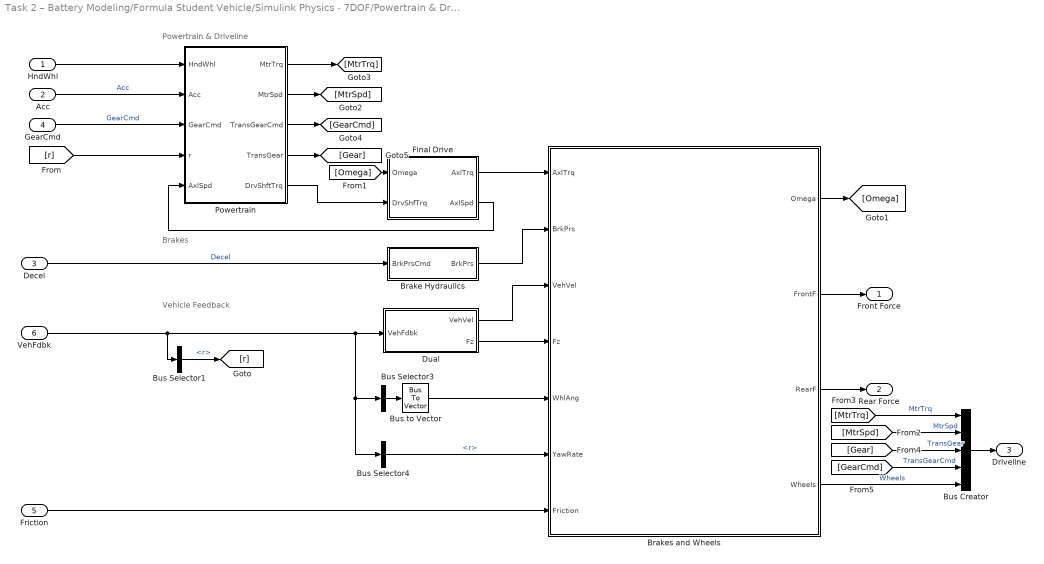
== system Task 2 – Battery Modeling/Formula Student Vehicle/Simulink Physics - 7DOF/Powertrain & Driveline ==
  note: Brakes
  note: Powertrain & Driveline
  note: Vehicle Feedback
  HndWhl : Inport
  Acc : Inport  Port=2
  Decel : Inport  Port=3
  GearCmd : Inport  Port=4
  Friction : Inport  Port=5
  VehFdbk : Inport  Port=6
  Brake Hydraulics : Subsystem
  Brakes and Wheels : Subsystem  TreatAsAtomicUnit=on
      mask Display: image('vdbslibwhls.png');
  Bus Creator : BusCreator  Inputs=5
  Bus Selector1 : BusSelector  OutputSignals=BdyFrm.Cg.AngVel.r
  Bus Selector3 : BusSelector  OutputSignals=BdyFrm.FrntAxl.Steer.WhlAngFL,BdyFrm.FrntAxl.Steer.WhlAngFR,BdyFrm.RearAxl.Steer.WhlAngRL,BdyFrm.RearAxl.Steer.WhlAngRR  OutputAsBus=on
  Bus Selector4 : BusSelector  OutputSignals=BdyFrm.Cg.AngVel.r
  Bus to Vector : BusToVector
  Dual : Subsystem  VariantControl=1
  Final Drive : Subsystem  Variant=on  VariantControlMode=label  VariantControl=Variant1  LabelModeActiveChoice=Direct
  Powertrain : Subsystem  Variant=on  VariantControlMode=label  VariantControl=Powertrain  LabelModeActiveChoice=EV4EM  EmptyChoice=on
  Front Force : Outport  VectorParamsAs1DForOutWhenUnconnected=off
  Rear Force : Outport  Port=2  VectorParamsAs1DForOutWhenUnconnected=off
  Driveline : Outport  Port=3  VectorParamsAs1DForOutWhenUnconnected=off
  wires:
  Bus Selector3/1 -> Bus to Vector/1
  [Omega] -> Final Drive/1(Omega)
  Decel/1 -> Brake Hydraulics/1(BrkPrsCmd)  "Decel"
  Friction/1 -> Brakes and Wheels/7(Friction)
  VehFdbk/1 -> Bus Selector1/1, Dual/1(VehFdbk), Bus Selector4/1, Bus Selector3/1
  Brakes and Wheels/1(Omega) -> [Omega]
  Brakes and Wheels/2(FrontF) -> Front Force/1
  Brakes and Wheels/3(RearF) -> Rear Force/1
  Bus to Vector/1 -> Brakes and Wheels/5(WhlAng)
  Bus Selector4/1 -> Brakes and Wheels/6(YawRate)  "<r>"
  Brake Hydraulics/1(BrkPrs) -> Brakes and Wheels/2(BrkPrs)
  Final Drive/1(AxlTrq) -> Brakes and Wheels/1(AxlTrq)
  Dual/1(VehVel) -> Brakes and Wheels/3(VehVel)
  Brakes and Wheels/4(Wheels) -> Bus Creator/5  "Wheels"
  Bus Creator/1 -> Driveline/1
  [MtrSpd] -> Bus Creator/2  "MtrSpd"
  [MtrTrq] -> Bus Creator/1  "MtrTrq"
  [Gear] -> Bus Creator/3  "TransGear"
  [GearCmd] -> Bus Creator/4  "TransGearCmd"
  Dual/2(Fz) -> Brakes and Wheels/4(Fz)
  Acc/1 -> Powertrain/2(Acc)  "Acc"
  GearCmd/1 -> Powertrain/3(GearCmd)  "GearCmd"
  Final Drive/2(AxlSpd) -> Powertrain/5(AxlSpd)
  Powertrain/1(MtrTrq) -> [MtrTrq]
  Powertrain/2(MtrSpd) -> [MtrSpd]
  Powertrain/3(TransGearCmd) -> [GearCmd]
  Powertrain/4(TransGear) -> [Gear]
  Powertrain/5(DrvShftTrq) -> Final Drive/2(DrvShfTrq)
  HndWhl/1 -> Powertrain/1(HndWhl)
  Bus Selector1/1 -> [r]  "<r>"
  [r] -> Powertrain/4(r)

== system Task 2 – Battery Modeling/Formula Student Vehicle/Simulink Physics - 7DOF/Steering ==
  HndWhl : Inport
  Kinematic Steering : vehdynlibsteering/Kinematic Steering  StrgType=Ackerman  StrgRatioType=Constant  Loc=Front  NrmlFctr=1  TrckWdth=VEH.TrackWidth  WhlBase=VEH.FrontAxlePositionfromCG+VEH.RearAxlePositionfromCG  Db=0  StrgRng=3*pi  StrgAngBpts="[-6.2832   -5.0265   -3.7699   -2.5133   -1.2566         0    1.2566    2.5133    3.7699    5.0265    6.2832]"  StrgRatioTbl=|  StrgRatio=10  PctAckIn=off  PctAck=100  PctAckTbl=ones(1,11)*100  StrgArmLngth=0.1  RckCsLngth=0.5  TieRodLngth=0.248128028933392  D=0.2  PnnRadius=0.0057  PnnRadiusTbl="[0.0055    0.0055    0.0056    0.0057    0.0057    0.0057    0.0057    0.0057    0.0056    0.0055    0.0055]"  RodLngth=0.1  ParaArmLngth=0.9  aMode=2
      | [13.5000   13.3750   13.2500   13.1250   13.0000   13.0000   13.0000   13.1250   13.2500   13.3750   13.5000
      | ]
  Mux : Mux  Inputs=2
  Normalized Steering : Gain  Gain=SteerLim*pi/180*10
  Terminator6 : Terminator
  FrntWhl : Outport  VectorParamsAs1DForOutWhenUnconnected=off
  wires:
  Kinematic Steering/1 -> Terminator6/1
  Kinematic Steering/2 -> Mux/1
  Kinematic Steering/3 -> Mux/2
  Mux/1 -> FrntWhl/1
  HndWhl/1 -> Normalized Steering/1
  Normalized Steering/1 -> Kinematic Steering/1

== system Task 2 – Battery Modeling/Formula Student Vehicle/Simulink Physics - 7DOF/Vehicle Body 3DOF Dual Track ==
  WhlAngF : Inport
  FwF : Inport  Port=2
  FwR : Inport  Port=3
  Terminator{1..5,7} (6 alike) : Terminator
  Vehicle Body 3DOF Dual Track : autolibshared/Vehicle Body 3DOF Single Track  trackMode=Dual  inputMode=External forces  frontSteerMode=on  rearSteerMode=off  windMode=off  muMode=off  extFMode=off  extMMode=off  htchFMode=off  htchMMode=off  extXo=off  extpsio=off  extxdoto=off  extro=off  extYo=off  extTamb=off  extydoto=off  aMode=2  NF=VEH.NumberOfWheelsPerAxle  NR=VEH.NumberOfWheelsPerAxle  m=VEH.Mass  a=VEH.FrontAxlePositionfromCG  b=VEH.RearAxlePositionfromCG  h=VEH.HeightCG/2  dh=1  hh=0.2  X_o=VEH.InitialLongPosition  xdot_o=VEH.InitialLongVel  CalphaMode=off  sigmaMode=on  d=0  hl=0  w=VEH.TrackWidth.*[1 1]  Cy_f=15000  Cy_r=35000  sigma_f=.1  sigma_r=.1  alpha_f_brk=[-.1 .1]  Cy_f_data=[2000, 3000, 4000, 5500, 7000, 9000, 7000, 5500, 4000, 3000, 2000]  alpha_r_brk=[-.1 .1]  Cy_r_data=[2000, 3000, 4000, 5500, 7000, 9000, 7000, 5500, 4000, 3000, 2000]  Y_o=VEH.InitialLatPosition  ydot_o=VEH.InitialLatVel  Izz=VEH.YawMomentInertia  psi_o=VEH.InitialYawAngle  r_o=VEH.InitialYawRate  Af=VEH.FrontalArea  Cd=VEH.DragCoefficient  Cl=.1  Cpm=.1  beta_w=[0 0.01:0.01:0.3]  Cs=[0 0.01:0.01:0.3]  Cym=[0 1e-6:0.01:0.3]  Pabs=101325  Tair=273  g=9.81  mu=1  xdot_tol=.01  Fznom=3800  Fxtire_sat=7e3*1e3  Fytire_sat=2e3*1e3  longOff=0  latOff=0  vertOff=.0112  wrapAng=off
  VehFdbk : Outport
  wires:
  Vehicle Body 3DOF Dual Track/6 -> Terminator3/1
  Vehicle Body 3DOF Dual Track/2 -> Terminator5/1
  Vehicle Body 3DOF Dual Track/3 -> Terminator1/1
  Vehicle Body 3DOF Dual Track/4 -> Terminator2/1
  Vehicle Body 3DOF Dual Track/7 -> Terminator4/1
  Vehicle Body 3DOF Dual Track/1 -> VehFdbk/1  "VehFdbk"
  Vehicle Body 3DOF Dual Track/5 -> Terminator7/1
  FwF/1 -> Vehicle Body 3DOF Dual Track/2
  WhlAngF/1 -> Vehicle Body 3DOF Dual Track/1
  FwR/1 -> Vehicle Body 3DOF Dual Track/3

== system Task 2 – Battery Modeling/Visualization/3D Visualization/Disabled ==

== system Task 2 – Battery Modeling/Visualization/3D Visualization/Enabled ==
  VehFdbk : Inport
  3D Visualization : Subsystem  Variant=on  VariantControl=Choice
  Cones : Subsystem  Variant=on  VariantControl=Choice
  wires:
  VehFdbk/1 -> 3D Visualization/1(VehFdbk)

== system Task 2 – Battery Modeling/Formula Student Vehicle/Simulink Physics - 7DOF/Environment/Ground Feedback ==
  note: 1) Add Subsystem or Model blocks as valid variant choices.
      | 2) You cannot connect blocks at this level. At simulation, connectivity is automatically
      | determined, based on the active variant and port name matching.
  Friction : Inport
  Constant : Subsystem  VariantControl=0
  Ground : Outport  VectorParamsAs1DForOutWhenUnconnected=off

== system Task 2 – Battery Modeling/Formula Student Vehicle/Simulink Physics - 7DOF/Powertrain & Driveline/Brake Hydraulics ==
  BrkPrsCmd : Inport
  Dead Zone : DeadZone  LowerValue=-inf  UpperValue=1e-3  ZeroCross=off
  Front Bias : Constant
  Gain4 : Gain  Gain=1e6
  Mux : Mux
  Product : Product
  Rear Bias : Constant  Value=.6
  Selector : Selector  InputPortWidth=1  IndexOptions=Index vector (dialog)  Indices=[1 1 1 1]  OutputSizes=1
  Valve : autolibutils/Cont LPF  wc=40*pi  AbsoluteTolerance=auto  aMode=2
  BrkPrs : Outport  VectorParamsAs1DForOutWhenUnconnected=off
  wires:
  BrkPrsCmd/1 -> Valve/1
  Valve/1 -> Dead Zone/1  "Flow"
  Gain4/1 -> BrkPrs/1
  Front Bias/1 -> Mux/2, Mux/1
  Rear Bias/1 -> Mux/3, Mux/4
  Product/1 -> Gain4/1
  Mux/1 -> Product/1
  Selector/1 -> Product/2
  Dead Zone/1 -> Selector/1
